simulink model "orig_exp_p"  (R2023a)
settings: Solver=ode4  StartTime=0.0  StopTime=10  FixedStep=0.001  RelTol=1e-3
settings Model: Creator=Anonymous  LastModifiedBy=Anonymous

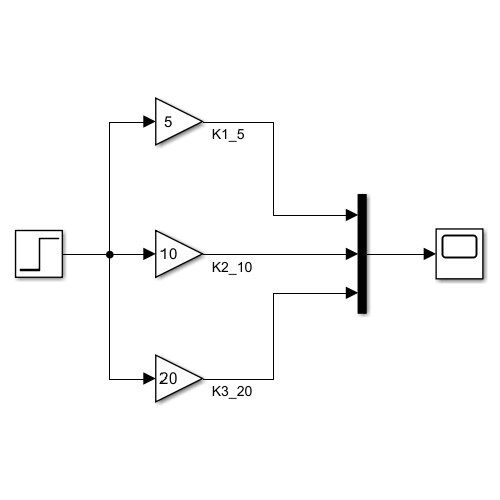
[thumbnail: Simulink's stored preview of the top-level diagram]
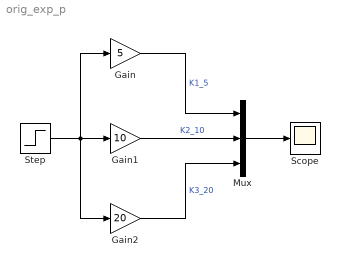
== system orig_exp_p ==
  Gain : Gain  Gain=5
  Gain1 : Gain  Gain=10
  Gain2 : Gain  Gain=20
  Mux : Mux  Inputs=3
  Scope : Scope
  Step : Step  SampleTime=0
  wires:
  Mux/1 -> Scope/1
  Gain2/1 -> Mux/3  "K3_20"
  Gain1/1 -> Mux/2  "K2_10"
  Gain/1 -> Mux/1  "K1_5"
  Step/1 -> Gain2/1, Gain1/1, Gain/1
